simulink model "motor_foc"  (R2022b)
settings: Solver=VariableStepAuto  StartTime=0.0  StopTime=10.0  RelTol=1e-3
values from neighbouring files (symbols this model uses):
  A = eye(4)    [sl_ekf.m]
libraries: spsThreePhaseVIMeasurementLib x4, spsPermanentMagnetSynchronousMachineLib x3, spsUniversalBridgeLib x3, spsDCVoltageSourceLib x2, ee_lib x1, spspowerguiLib x1
settings Model: Creator=15403  LastModifiedBy=15403

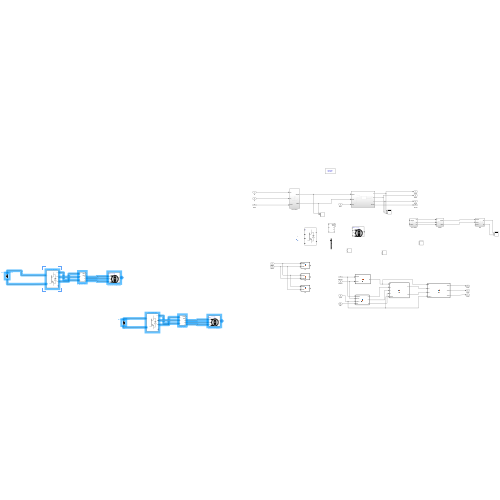
[thumbnail: Simulink's stored preview of the top-level diagram]
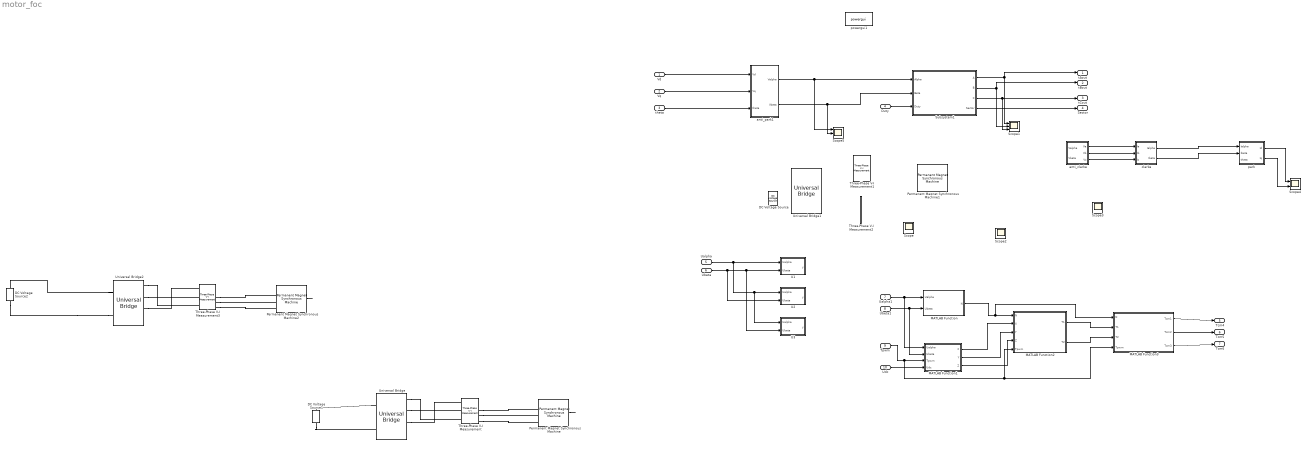
== system motor_foc ==
  Vd : Inport
  Vq : Inport  Port=2
  theta : Inport  Port=3
  Duty : Inport  Port=4
  Ualpha : Inport  Port=5
  Ubeta : Inport  Port=6
  Ualpha1 : Inport  Port=7
  Ubeta1 : Inport  Port=8
  Tpwm : Inport  Port=9
  Udc : Inport  Port=10
  DC Voltage Source : ee_lib/Additional Components/SPICE Sources/DC Voltage Source  DC=24 V
  DC Voltage Source1 : spsDCVoltageSourceLib/DC Voltage Source  Amplitude=100  Measurements=None
  DC Voltage Source2 : spsDCVoltageSourceLib/DC Voltage Source  Amplitude=100  Measurements=None
  MATLAB Function : MATLAB Function  TreatAsAtomicUnit=on
  MATLAB Function1 : MATLAB Function  TreatAsAtomicUnit=on
  MATLAB Function2 : MATLAB Function  TreatAsAtomicUnit=on
  MATLAB Function3 : MATLAB Function  TreatAsAtomicUnit=on
  Permanent Magnet Synchronous Machine : spsPermanentMagnetSynchronousMachineLib/Permanent Magnet Synchronous Machine  NbPhases=3  FluxDistribution=Sinusoidal  RotorType=Round  MechanicalLoad=Torque Tm  PresetModel=No  ShowDetailedParameters=on  MeasurementBus=off  Resistance=0.1478  Inductance=8.5e-3  dqInductances=[8.5e-3,8.5e-3]  La=0.00025951  MachineConstant=Flux linkage established by magnets (V.s)  Flux=0.142879  VoltageCst=51.8308  TorqueCst=0.42864  Flat=120  Mechanical=[0.000621417 0.000303448 2]  PolePairs=4  InitialConditions=[0,0, 0,0]  InitialConditions5ph=[0 0 0 0 0 0]  RefAngle=90 degrees behind phase A axis (modified Park)  IterativeDiscreteModel=Trapezoidal non iterative  TsBlock=-1  TsPowergui=0
  Permanent Magnet Synchronous Machine1 : spsPermanentMagnetSynchronousMachineLib/Permanent Magnet Synchronous Machine  NbPhases=3  FluxDistribution=Sinusoidal  RotorType=Round  MechanicalLoad=Torque Tm  PresetModel=No  ShowDetailedParameters=on  MeasurementBus=off  Resistance=0.1478  Inductance=8.5e-3  dqInductances=[8.5e-3,8.5e-3]  La=0.00025951  MachineConstant=Flux linkage established by magnets (V.s)  Flux=0.142879  VoltageCst=51.8308  TorqueCst=0.42864  Flat=120  Mechanical=[0.000621417 0.000303448 2]  PolePairs=4  InitialConditions=[0,0, 0,0]  InitialConditions5ph=[0 0 0 0 0 0]  RefAngle=90 degrees behind phase A axis (modified Park)  IterativeDiscreteModel=Trapezoidal non iterative  TsBlock=-1  TsPowergui=0
  Permanent Magnet Synchronous Machine2 : spsPermanentMagnetSynchronousMachineLib/Permanent Magnet Synchronous Machine  NbPhases=3  FluxDistribution=Sinusoidal  RotorType=Round  MechanicalLoad=Torque Tm  PresetModel=No  ShowDetailedParameters=on  MeasurementBus=off  Resistance=0.1478  Inductance=8.5e-3  dqInductances=[8.5e-3,8.5e-3]  La=0.00025951  MachineConstant=Flux linkage established by magnets (V.s)  Flux=0.142879  VoltageCst=51.8308  TorqueCst=0.42864  Flat=120  Mechanical=[0.000621417 0.000303448 2]  PolePairs=4  InitialConditions=[0,0, 0,0]  InitialConditions5ph=[0 0 0 0 0 0]  RefAngle=90 degrees behind phase A axis (modified Park)  IterativeDiscreteModel=Trapezoidal non iterative  TsBlock=-1  TsPowergui=0
  Scope : Scope  NumInputPorts=2
  Scope1 : Scope  NumInputPorts=3
  Scope2 : Scope  NumInputPorts=3
  Scope3 : Scope  NumInputPorts=2
  Scope4 : Scope  NumInputPorts=2
  Scope5 : Scope  NumInputPorts=3
  Subsystem1 : Subsystem
  Three-Phase V-I Measurement : spsThreePhaseVIMeasurementLib/Three-Phase V-I Measurement  VoltageMeasurement=phase-to-ground  SetLabelV=off  LabelV=Vabc  Vpu=off  VpuLL=off  CurrentMeasurement=yes  SetLabelI=off  LabelI=Iabc  Ipu=off  Pbase=100e6  Vbase=500e3  OutputType=Complex  PhasorSimulation=off  PSBequivalent=0
  Three-Phase V-I Measurement1 : spsThreePhaseVIMeasurementLib/Three-Phase V-I Measurement  VoltageMeasurement=phase-to-ground  SetLabelV=off  LabelV=Vabc  Vpu=off  VpuLL=off  CurrentMeasurement=yes  SetLabelI=off  LabelI=Iabc  Ipu=off  Pbase=100e6  Vbase=500e3  OutputType=Complex  PhasorSimulation=off  PSBequivalent=0
  Three-Phase V-I Measurement2 : spsThreePhaseVIMeasurementLib/Three-Phase V-I Measurement  VoltageMeasurement=no  SetLabelV=off  LabelV=Vabc  Vpu=off  VpuLL=off  CurrentMeasurement=no  SetLabelI=off  LabelI=Iabc  Ipu=off  Pbase=100e6  Vbase=500e3  OutputType=Complex  PhasorSimulation=off  PSBequivalent=0
  Three-Phase V-I Measurement3 : spsThreePhaseVIMeasurementLib/Three-Phase V-I Measurement  VoltageMeasurement=phase-to-ground  SetLabelV=off  LabelV=Vabc  Vpu=off  VpuLL=off  CurrentMeasurement=yes  SetLabelI=off  LabelI=Iabc  Ipu=off  Pbase=100e6  Vbase=500e3  OutputType=Complex  PhasorSimulation=off  PSBequivalent=0
  U1 : MATLAB Function  TreatAsAtomicUnit=on
  U2 : MATLAB Function  TreatAsAtomicUnit=on
  U3 : MATLAB Function  TreatAsAtomicUnit=on
  Universal Bridge : spsUniversalBridgeLib/Universal Bridge  Arms=3  SnubberResistance=1e5  SnubberCapacitance=inf  Device=IGBT / Diodes  Ron=1e-3  Lon=0  ForwardVoltages="[  0  0  ]"  ForwardVoltage=0  GTOparameters=[ 10e-6 , 20e-6 ]  IGBTparameters=[ 1e-6 , 2e-6 ]  Measurements=None  Measurements_2=None  converterType=Rectifier
  Universal Bridge1 : spsUniversalBridgeLib/Universal Bridge  Arms=3  SnubberResistance=1e5  SnubberCapacitance=inf  Device=IGBT / Diodes  Ron=1e-3  Lon=0  ForwardVoltages="[  0  0  ]"  ForwardVoltage=0  GTOparameters=[ 10e-6 , 20e-6 ]  IGBTparameters=[ 1e-6 , 2e-6 ]  Measurements=None  Measurements_2=None  converterType=Rectifier
  Universal Bridge2 : spsUniversalBridgeLib/Universal Bridge  Arms=3  SnubberResistance=1e5  SnubberCapacitance=inf  Device=IGBT / Diodes  Ron=1e-3  Lon=0  ForwardVoltages="[  0  0  ]"  ForwardVoltage=0  GTOparameters=[ 10e-6 , 20e-6 ]  IGBTparameters=[ 1e-6 , 2e-6 ]  Measurements=None  Measurements_2=None  converterType=Rectifier
  anti_clarke : Subsystem
  anti_park1 : Subsystem
  clarke : Subsystem
  park : Subsystem
  powergui1 : spspowerguiLib/powergui  Priority=1  SimulationMode=Discrete  SampleTime=50e-6  frequency=60  Iterations=50  frequencyindice=60  Pbase=100e6  ErrMax=1e-4  UnitsV=kV  UnitsW=MW  buscounter=0  FunctionMessages=off  echomessages=off  EnableUseOfTLC=off  CurrentSourceSwitches=off  DisableSnubberDevices=off  DisableRonSwitches=off  DisableVfSwitches=off  DisplayEquations=off  AutomaticDiscreteSolvers=off  SolverType=Tustin/Backward Euler (TBE)  Interpol=off  ExternalGateDelay=off  methode=off  Ts=100  x0status=blocks  SPID=on  SwTol=0  HookPort=off  NonlinearTolerance=1e-4  nMaxIteration=100  ContinueOnMaxIteration=off  RestoreLinks=warning  ResistiveCurrentMeasurement=off  Frange=[0:2:500]  Ylog=off  Xlog=on  ShowGrid=off  save=off  variable=ZData  structure=0  ZoomFFT=off  StartTime=0.0  cycles=1  DisplayStyle=1  fundamental=60  FreqAxis=off  MaxFrequency=1000  frequencyindicesteady=1  RmsSteady=1  display=off
  tAout : Outport
  tBout : Outport  Port=2
  tCout : Outport  Port=3
  Sector : Outport  Port=4
  Tcm4 : Outport  Port=5
  Tcm5 : Outport  Port=6
  Tcm6 : Outport  Port=7
  wires:
  MATLAB Function3/3(Tcm3) -> Tcm6/1
  Udc/1 -> MATLAB Function1/4(Udc)
  Subsystem1/1(A) -> Scope1/1, tAout/1
  anti_park1/2(Vbeta) -> Scope5/2, Subsystem1/2(Beta)
  anti_clarke/3(Vc) -> clarke/3(Ic)
  Vq/1 -> anti_park1/2(Vq)
  theta/1 -> anti_park1/3(theta)
  MATLAB Function3/2(Tcm2) -> Tcm5/1
  MATLAB Function1/2(Y) -> MATLAB Function2/3(Y)
  MATLAB Function3/1(Tcm1) -> Tcm4/1
  Ubeta/1 -> U2/2(Ubeta), U3/2(Ubeta), U1/2(Ubeta)
  Tpwm/1 -> MATLAB Function3/4(Tpwm), MATLAB Function2/5(Tpwm), MATLAB Function1/3(Tpwm)
  Subsystem1/2(B) -> Scope1/2, tBout/1
  anti_park1/1(Valpha) -> Scope5/1, Subsystem1/1(Alpha)
  park/1(Id) -> Scope4/1
  MATLAB Function/1(N) -> MATLAB Function3/1(N), MATLAB Function2/1(N)
  MATLAB Function1/1(X) -> MATLAB Function2/2(X)
  Subsystem1/3(C) -> Scope1/3, tCout/1
  MATLAB Function2/2(T2) -> MATLAB Function3/3(T2)
  Ualpha1/1 -> MATLAB Function1/1(Ualpha), MATLAB Function/1(Ualpha)
  Ualpha/1 -> U3/1(Ualpha), U2/1(Ualpha), U1/1(Ualpha)
  anti_clarke/1(Va) -> clarke/1(Ia)
  clarke/2(Ibeta) -> park/2(Ibeta)
  clarke/1(Ialpha) -> park/1(Ialpha)
  MATLAB Function1/3(Z) -> MATLAB Function2/4(Z)
  park/2(Iq) -> Scope4/2
  anti_clarke/2(Vb) -> clarke/2(Ib)
  Subsystem1/4(Sector) -> Sector/1
  MATLAB Function2/1(T1) -> MATLAB Function3/2(T1)
  Duty/1 -> Subsystem1/3(Duty)
  Vd/1 -> anti_park1/1(Vd)
  Ubeta1/1 -> MATLAB Function1/2(Ubeta), MATLAB Function/2(Ubeta)
  Permanent Magnet Synchronous Machine/1 -> ?
  Permanent Magnet Synchronous Machine2/1 -> ?
  connections:
  Universal Bridge/LConn3 -- Three-Phase V-I Measurement/LConn3
  DC Voltage Source1/RConn1 -- Universal Bridge/RConn1
  Universal Bridge/RConn2 -- DC Voltage Source1/LConn1
  Universal Bridge/LConn1 -- Three-Phase V-I Measurement/LConn1
  Universal Bridge/LConn2 -- Three-Phase V-I Measurement/LConn2
  Three-Phase V-I Measurement/RConn1 -- Permanent Magnet Synchronous Machine/LConn1
  Three-Phase V-I Measurement/RConn3 -- Permanent Magnet Synchronous Machine/LConn3
  Three-Phase V-I Measurement/RConn2 -- Permanent Magnet Synchronous Machine/LConn2
  Universal Bridge2/LConn3 -- Three-Phase V-I Measurement3/LConn3
  DC Voltage Source2/RConn1 -- Universal Bridge2/RConn1
  Universal Bridge2/RConn2 -- DC Voltage Source2/LConn1
  Universal Bridge2/LConn1 -- Three-Phase V-I Measurement3/LConn1
  Universal Bridge2/LConn2 -- Three-Phase V-I Measurement3/LConn2
  Three-Phase V-I Measurement3/RConn1 -- Permanent Magnet Synchronous Machine2/LConn1
  Three-Phase V-I Measurement3/RConn3 -- Permanent Magnet Synchronous Machine2/LConn3
  Three-Phase V-I Measurement3/RConn2 -- Permanent Magnet Synchronous Machine2/LConn2

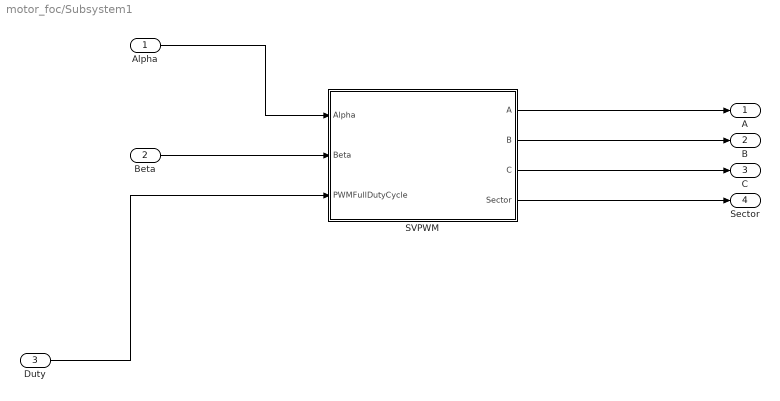
== system motor_foc/Subsystem1 ==
  Alpha : Inport
  Beta : Inport  Port=2
  Duty : Inport  Port=3
  SVPWM : MATLAB Function  TreatAsAtomicUnit=on
  A : Outport
  B : Outport  Port=2
  C : Outport  Port=3
  Sector : Outport  Port=4
  wires:
  SVPWM/1(A) -> A/1
  Duty/1 -> SVPWM/3(PWMFullDutyCycle)
  Alpha/1 -> SVPWM/1(Alpha)
  Beta/1 -> SVPWM/2(Beta)
  SVPWM/3(C) -> C/1
  SVPWM/4(Sector) -> Sector/1
  SVPWM/2(B) -> B/1

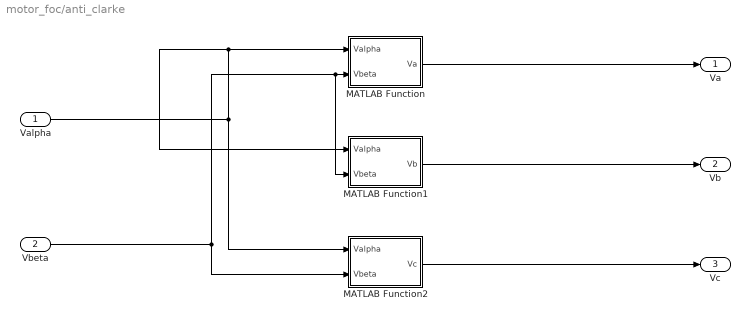
== system motor_foc/anti_clarke ==
  " Valpha" : Inport
  Vbeta : Inport  Port=2
  MATLAB Function : MATLAB Function  TreatAsAtomicUnit=on
  MATLAB Function1 : MATLAB Function  TreatAsAtomicUnit=on
  MATLAB Function2 : MATLAB Function  TreatAsAtomicUnit=on
  Va : Outport
  Vb : Outport  Port=2
  Vc : Outport  Port=3
  wires:
  MATLAB Function/1(Va) -> Va/1
  Vbeta/1 -> MATLAB Function1/2(Vbeta), MATLAB Function/2(Vbeta), MATLAB Function2/2(Vbeta)
  " Valpha"/1 -> MATLAB Function/1(Valpha), MATLAB Function1/1(Valpha), MATLAB Function2/1(Valpha)
  MATLAB Function1/1(Vb) -> Vb/1
  MATLAB Function2/1(Vc) -> Vc/1

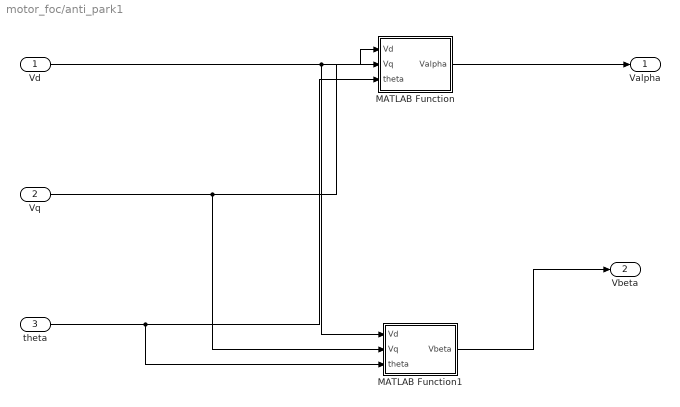
== system motor_foc/anti_park1 ==
  Vd : Inport
  Vq : Inport  Port=2
  theta : Inport  Port=3
  MATLAB Function : MATLAB Function  TreatAsAtomicUnit=on
  MATLAB Function1 : MATLAB Function  TreatAsAtomicUnit=on
  Valpha : Outport
  Vbeta : Outport  Port=2
  wires:
  MATLAB Function/1(Valpha) -> Valpha/1
  MATLAB Function1/1(Vbeta) -> Vbeta/1
  Vd/1 -> MATLAB Function/1(Vd), MATLAB Function1/1(Vd)
  Vq/1 -> MATLAB Function/2(Vq), MATLAB Function1/2(Vq)
  theta/1 -> MATLAB Function/3(theta), MATLAB Function1/3(theta)

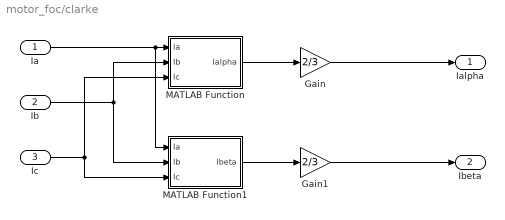
== system motor_foc/clarke ==
  Ia : Inport
  Ib : Inport  Port=2
  Ic : Inport  Port=3
  Gain : Gain  Gain=2/3  OutDataTypeStr=single
  Gain1 : Gain  Gain=2/3  OutDataTypeStr=single
  MATLAB Function : MATLAB Function  TreatAsAtomicUnit=on
  MATLAB Function1 : MATLAB Function  TreatAsAtomicUnit=on
  Ialpha : Outport
  Ibeta : Outport  Port=2
  wires:
  Ia/1 -> MATLAB Function1/1(Ia), MATLAB Function/1(Ia)
  MATLAB Function/1(Ialpha) -> Gain/1
  Gain1/1 -> Ibeta/1
  Ib/1 -> MATLAB Function1/2(Ib), MATLAB Function/2(Ib)
  Ic/1 -> MATLAB Function/3(Ic), MATLAB Function1/3(Ic)
  MATLAB Function1/1(Ibeta) -> Gain1/1
  Gain/1 -> Ialpha/1

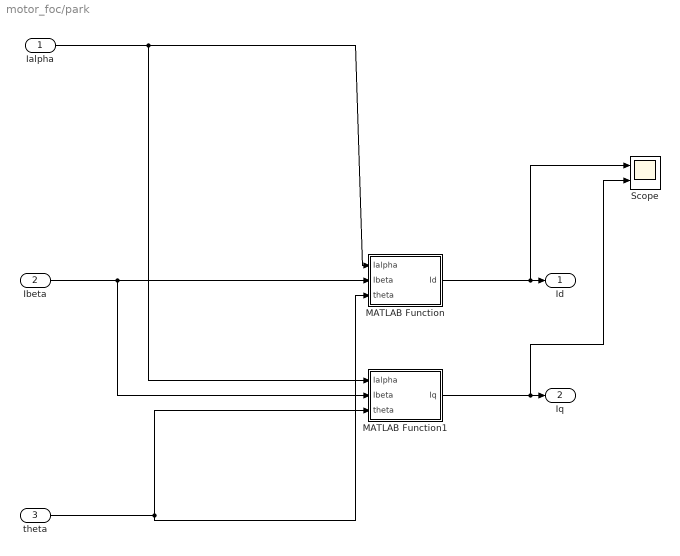
== system motor_foc/park ==
  Ialpha : Inport
  Ibeta : Inport  Port=2
  theta : Inport  Port=3
  MATLAB Function : MATLAB Function  TreatAsAtomicUnit=on
  MATLAB Function1 : MATLAB Function  TreatAsAtomicUnit=on
  Scope : Scope  NumInputPorts=2
  Id : Outport
  Iq : Outport  Port=2
  wires:
  theta/1 -> MATLAB Function/3(theta), MATLAB Function1/3(theta)
  Ibeta/1 -> MATLAB Function/2(Ibeta), MATLAB Function1/2(Ibeta)
  MATLAB Function1/1(Iq) -> Scope/2, Iq/1
  MATLAB Function/1(Id) -> Scope/1, Id/1
  Ialpha/1 -> MATLAB Function/1(Ialpha), MATLAB Function1/1(Ialpha)

== matlab function motor_foc/U2 ==
  data: Ualpha input; y output; Ubeta input
function y = fcn(Ualpha, Ubeta)

y = sqrt(3) * Ualpha +- Ubeta;

== matlab function motor_foc/U3 ==
  data: Ualpha input; y output; Ubeta input
function y = fcn(Ualpha, Ubeta)

y = -sqrt(3) * Ualpha - Ubeta;

== matlab function motor_foc/anti_park1/MATLAB Function ==
  data: Vd input; Valpha output; Vq input; theta input
function Valpha = fcn(Vd, Vq, theta)

Valpha = Vd * cos(theta) - Vq * sin(theta);

== matlab function motor_foc/anti_park1/MATLAB Function1 ==
  data: Vd input; Vbeta output; Vq input; theta input
function Vbeta = fcn(Vd, Vq, theta)

Vbeta = Vd * sin(theta) + Vq * cos(theta);

== matlab function motor_foc/MATLAB Function ==
  data: Ualpha input; N output; Ubeta input
function N = fcn(Ualpha, Ubeta)

U1 = Ubeta;
U2 = sqrt(3) * Ualpha - Ubeta;
U3 = -sqrt(3) * Ualpha - Ubeta;
A = 0;
B = 0;
C = 0;

if U1 > 0
    A = 1;
else
    A = 0;
end

if U2 > 0
    B = 1;
else
    B = 0;
end

if U3 > 0
    C = 1;
else
    C = 0;
end

N = A + 2 * B + 4 * C;

== matlab function motor_foc/clarke/MATLAB Function ==
  data: Ia input; Ialpha output; Ib input; Ic input
function Ialpha = fcn(Ia, Ib, Ic)

Ialpha = 3/2 * Ia;

== matlab function motor_foc/clarke/MATLAB Function1 ==
  data: Ia input; Ibeta output; Ib input; Ic input
function Ibeta = fcn( Ia, Ib, Ic)

Ibeta = sqrt(3)/2 * (Ia + 2 * Ib);

== matlab function motor_foc/park/MATLAB Function ==
  data: Ialpha input; Id output; Ibeta input; theta input
function Id = fcn(Ialpha, Ibeta, theta)

Id = Ialpha * cos(theta) + Ibeta * sin(theta);

== matlab function motor_foc/park/MATLAB Function1 ==
  data: Ialpha input; Iq output; Ibeta input; theta input
function Iq = fcn(Ialpha, Ibeta, theta)
Iq = -Ialpha * sin(theta) + Ibeta * cos(theta);

== matlab function motor_foc/MATLAB Function1 ==
  data: Ualpha input; Ubeta input; Tpwm input; Udc input; X output; Y output; Z output
function [X, Y, Z] = fcn(Ualpha, Ubeta, Tpwm, Udc)

X = sqrt(3) * Tpwm * Ubeta / Udc;
Y = sqrt(3) * Tpwm / Udc * (sqrt(3) / 2 * Ualpha + 1 / 2 * Ubeta);
Z = sqrt(3) * Tpwm / Udc * (-sqrt(3) / 2 * Ualpha + 1 / 2 * Ubeta);

== matlab function motor_foc/MATLAB Function2 ==
  data: N input; T1 output; X input; Y input; Z input; Tpwm input; T2 output
function [T1, T2] = fcn(N, X, Y, Z, Tpwm)

if N == 1
    T1 = Z;
    T2 = Y;
elseif N == 2
    T1 = Y;
    T2 = -X;
elseif N == 3
    T1 = -Z;
    T2 = X;
elseif N == 4
    T1 = -X;
    T2 = Z;
elseif N == 5
    T1 = X;
    T2 = -Y;
elseif N == 6
    T1 = -Y;
    T2 = -Z;
end

== matlab function motor_foc/MATLAB Function3 ==
  data: N input; Tcm1 output; T1 input; T2 input; Tpwm input; Tcm2 output; Tcm3 output
function [Tcm1, Tcm2, Tcm3] = fcn(N, T1, T2, Tpwm)

if N == 1
    Tcm1 = (Tpwm + T1 - T2) / 4;
    Tcm2 = (Tpwm - T1 - T2) / 4;
    Tcm3 = (Tpwm + T1 + T2) / 4;
elseif N == 2
    Tcm1 = (Tpwm - T1 - T2) / 4;
    Tcm2 = (Tpwm + T1 + T2) / 4;
    Tcm3 = (Tpwm + T1 - T2) / 4;
elseif N == 3
    Tcm1 = (Tpwm - T1 - T2) / 4;
    Tcm2 = (Tpwm + T1 - T2) / 4;
    Tcm3 = (Tpwm + T1 + T2) / 4;
elseif N == 4
    Tcm1 = (Tpwm + T1 + T2) / 4;
    Tcm2 = (Tpwm + T1 - T2) / 4;
    Tcm3 = (Tpwm - T1 - T2) / 4;
elseif N == 5
    Tcm1 = (Tpwm + T1 + T2) / 4;
    Tcm2 = (Tpwm - T1 - T2) / 4;
    Tcm3 = (Tpwm + T1 - T2) / 4;
elseif N == 6
    Tcm1 = (Tpwm + T1 - T2) / 4;
    Tcm2 = (Tpwm + T1 + T2) / 4;
    Tcm3 = (Tpwm - T1 - T2) / 4;
end

== matlab function motor_foc/anti_clarke/MATLAB Function ==
  data: Va output; Valpha input; Vbeta input
function Va = fcn(Valpha, Vbeta)

Va = Valpha;

== matlab function motor_foc/anti_clarke/MATLAB Function1 ==
  data: Valpha input; Vb output; Vbeta input
function Vb = fcn(Valpha, Vbeta)

Vb = -Valpha * 1/2 + Vbeta * sqrt(3) / 2;

== matlab function motor_foc/anti_clarke/MATLAB Function2 ==
  data: Valpha input; Vc output; Vbeta input
function Vc = fcn(Valpha, Vbeta)
Vc = -Valpha * 1/2 - Vbeta * sqrt(3) / 2;

== matlab function motor_foc/Subsystem1/SVPWM ==
  data: Alpha input; A output; B output; C output; Sector output; Beta input; PWMFullDutyCycle input
function [A, B, C, Sector] = fcn(Alpha, Beta, PWMFullDutyCycle)

% 初始化变量
A = single(0);
B = single(0);
C = single(0);                                  
Sector = 0;
ONE_BY_SQRT3 = 0.57735026919;
TWO_BY_SQRT3 = (2.0 * 0.57735026919);

% 扇区判断
if Beta >= 0.0
    if Alpha >= 0.0
        if (ONE_BY_SQRT3 * Beta) > Alpha
            Sector = 2;
        else
            Sector = 1;
        end
    else
        if -ONE_BY_SQRT3 * Beta > Alpha
            Sector = 3;
        else
            Sector = 2;
        end
    end
else
    if Alpha >= 0.0
        if -ONE_BY_SQRT3 * Beta > Alpha
            Sector = 5;
        else
            Sector = 6;
        end

    else
        if ONE_BY_SQRT3 * Beta > Alpha
            Sector = 4;
        else
            Sector = 5;
        end
    end
end


switch Sector
    case 1
        t1 = (Alpha - ONE_BY_SQRT3 * Beta) * PWMFullDutyCycle;
        t2 = (TWO_BY_SQRT3 * Beta) * PWMFullDutyCycle;

        A = (PWMFullDutyCycle + t1 + t2) / 2;
        B = A - t1;
        C = B - t2;
    case 2
		t2 = (Alpha + ONE_BY_SQRT3 * Beta) * PWMFullDutyCycle;
		t3 = (-Alpha + ONE_BY_SQRT3 * Beta) * PWMFullDutyCycle;

		B = (PWMFullDutyCycle + t2 + t3) / 2;
		A = B - t3;
		C = A - t2;
        
    case 3
        t3 = (TWO_BY_SQRT3 * Beta) * PWMFullDutyCycle;
		t4 = (-Alpha - ONE_BY_SQRT3 * Beta) * PWMFullDutyCycle;

		B = (PWMFullDutyCycle + t3 + t4) / 2;
		C = B - t3;
		A = C - t4;

    case 4
		t4 = (-Alpha + ONE_BY_SQRT3 * Beta) * PWMFullDutyCycle;
		t5 = (-TWO_BY_SQRT3 * Beta) * PWMFullDutyCycle;

		C = (PWMFullDutyCycle + t4 + t5) / 2;
		B = C - t5;
		A = B - t4;
    case 5
        t5 = (-Alpha - ONE_BY_SQRT3 * Beta) * PWMFullDutyCycle;
		t6 = (Alpha - ONE_BY_SQRT3 * Beta) * PWMFullDutyCycle;

		C = (PWMFullDutyCycle + t5 + t6) / 2;
		A = C - t5;
		B = A - t6;

    case 6
		t6 = (-TWO_BY_SQRT3 * Beta) * PWMFullDutyCycle;
		t1 = (Alpha + ONE_BY_SQRT3 * Beta) * PWMFullDutyCycle;

		A = (PWMFullDutyCycle + t6 + t1) / 2;
		C = A - t1;
		B = C - t6;
end

== matlab function motor_foc/U1 ==
  data: Ualpha input; y output; Ubeta input
function y = fcn(Ualpha, Ubeta)

y = Ubeta;
